simulink model "orig_exp_frequency"  (R2023a)
settings: Solver=ode4  StartTime=0.0  StopTime=90  FixedStep=0.001  RelTol=1e-3
settings Model: Creator=Anonymous  LastModifiedBy=Anonymous

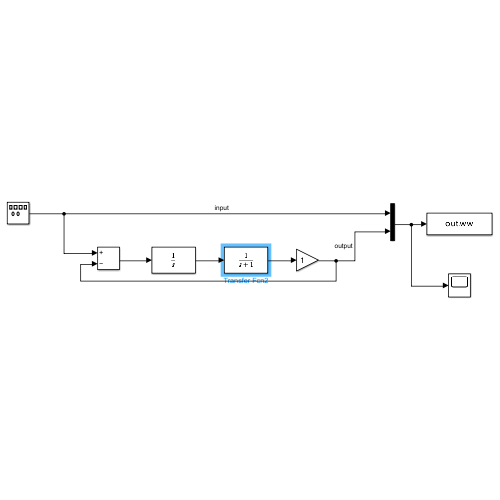
[thumbnail: Simulink's stored preview of the top-level diagram]
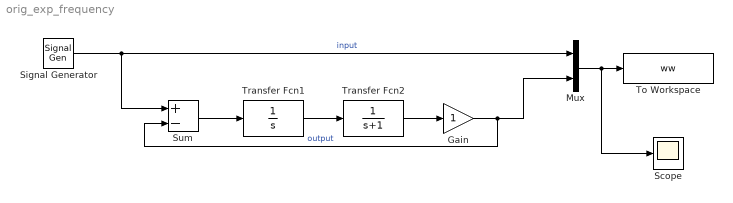
== system orig_exp_frequency ==
  Gain : Gain
  Mux : Mux  Inputs=2
  Scope : Scope
  Signal Generator : SignalGenerator  Frequency=0.707  Units=rad/sec
  Sum : Sum  Inputs=+-
  To Workspace : ToWorkspace  VariableName=ww  SaveFormat=Structure With Time  SampleTime=-1
  Transfer Fcn1 : TransferFcn  Numerator=1  Denominator=[1 0]
  Transfer Fcn2 : TransferFcn  Numerator=1  Denominator=[1 1]
  wires:
  Mux/1 -> To Workspace/1, Scope/1
  Gain/1 -> Mux/2, Sum/2  "output"
  Transfer Fcn2/1 -> Gain/1
  Transfer Fcn1/1 -> Transfer Fcn2/1
  Sum/1 -> Transfer Fcn1/1
  Signal Generator/1 -> Mux/1, Sum/1  "input"
